simulink model "F104_FC2_sim"  (R2026b)
settings: Solver=ode45  StopTime=200  MaxStep=0.01  RelTol=1e-6  AbsTol=1e-8
undefined symbols (not defined in the file or in its folder): A, alt_m, B, C, D, pos_scale, thetae, V_ms, x0
libraries: aerolibsim3d x2, sim3dlib x1
settings Model: Creator=tensei  LastModifiedBy=tensei

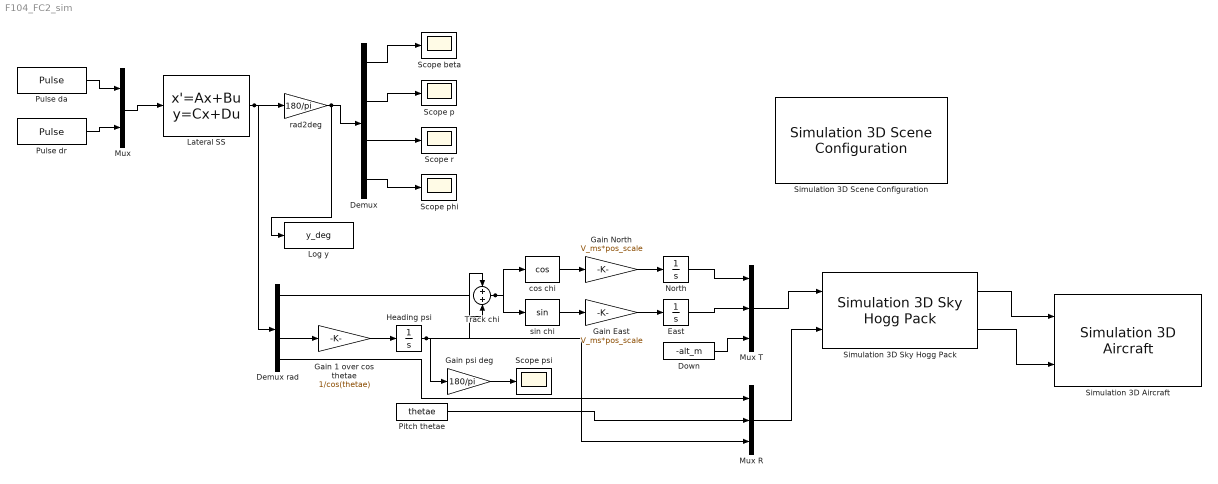
== system F104_FC2_sim ==
  Demux : Demux
  Demux rad : Demux
  Down : Constant  Value=-alt_m
  East : Integrator
  Gain 1 over cos thetae : Gain  Gain=1/cos(thetae)
  Gain East : Gain  Gain=V_ms*pos_scale
  Gain North : Gain  Gain=V_ms*pos_scale
  Gain psi deg : Gain  Gain=180/pi
  Heading psi : Integrator
  Lateral SS : StateSpace  A=A  B=B  C=C  D=D  InitialCondition=x0
  Log y : ToWorkspace  VariableName=y_deg  SampleTime=-1
  Mux : Mux  Inputs=2
  Mux R : Mux  Inputs=3
  Mux T : Mux  Inputs=3
  North : Integrator
  Pitch thetae : Constant  Value=thetae
  Pulse da : DiscretePulseGenerator  PulseType=Time based  Amplitude=0  Period=100
  Pulse dr : DiscretePulseGenerator  PulseType=Time based  Amplitude=0.034906  Period=100
  Scope beta : Scope
  Scope p : Scope
  Scope phi : Scope
  Scope psi : Scope
  Scope r : Scope
  Simulation 3D Aircraft : aerolibsim3d/Simulation 3D Aircraft  Priority=-1  Mesh=Sky Hogg  MeshPath=/MathWorksAerospaceContent/Vehicles/Aircraft/Custom/Mesh/SK_HL20.SK_HL20  MeshPathAT=/MathWorksAerospaceContent/Vehicles/Aircraft/AirTransport/Mesh/SK_AirTransport.SK_AirTransport  MeshPathGA=/MathWorksAerospaceContent/Vehicles/Aircraft/GeneralAviation/Mesh/SK_GeneralAviation.SK_GeneralAviation  AircraftColor=Red  ActorName=SimulinkVehicle1  ShowICs=on  Translation=[0 0 0; zeros(10,3)]  Rotation=[0 0 0; zeros(10,3)]  ScaleInputPort=Dialog  Scale=[1 1 1]  InitialScale=[1 1 1]  IsGHSensorEnabled=off  AreGHRaysVisible=off  IsOutputReshapeEnabled=off  GHRayLength=1524  GHBodyOffset=0.90  GHFrontTireRadius=0.21  GHLeftTireRadius=0.21  GHRightTireRadius=0.21  WoWSensorTolerance=0.05  LightsConfig=Automatic lights  LandingLightIntensity=300000  LandingLightConeAngle=15  CustomLeftLandingLightLocation=[0 0 0]  CustomLeftLandingLightOrientation=[0 0 0]  CustomRightLandingLightLocation=[0 0 0]  CustomRightLandingLightOrientation=[0 0 0]  TaxiLightIntensity=150000  TaxiLightConeAngle=36  CustomTaxiLightLocation=[0 0 0]  CustomTaxiLightOrientation=[0 0 0]  NavLightIntensity=500  PositionLightIntensity=500  StrobeLightIntensity=5000  WingtipStrobePeriod=1.5  WingtipStrobePulseWidth=6  TailStrobePeriod=1.5  TailStrobePulseWidth=6  BeaconLightIntensity=4000  BeaconPeriod=1.5  BeaconPulseWidth=10  SampleTime=-1  ActorType=SimulinkVehicle  ID=1  aMode=0  ActorTag=SimulinkVehicle1
  Simulation 3D Scene Configuration : sim3dlib/Simulation 3D Scene Configuration  Priority=0  EnableWindow=on  ViewerType=Default Viewer  ProjectFormat=Default Scenes  SceneDesc=Empty scene  ProjectName=/usr/local/MATLAB/R2026b/toolbox/shared/sim3d_projects/automotive_project_linux/UE/LinuxNoEditor/VehicleSimulation.sh  ScenePath=/Game/Maps/HwStrght  EnableOpenDRIVE=off  vehTagList={'Custom';'Scene Origin';'SimulinkVehicle1'}  vehTag=SimulinkVehicle1  AttachedCameraRelativeTranslation=[0 0 0]  FreeCameraDefaultInitialTranslation=[-6, 0, 2]  AttachedCameraRelativeRotation=[0, -15, 0]  FreeCameraDefaultInitialRotation=[0, -15, 0]  ViewpointName=Custom  FreeCameraInitialTranslation=[0, 0, 0]  FreeCameraInitialRotation=[0, 0, 0]  OpVisEn=off  Ts=.1  EnableRemoteAccess=off  SimulationMode=CoSimulation  SimulateUsing=Interpreted execution  EnableAnimationRecording=off  OverrideDefaultRecording=off  AnimationRecordingFileName=sim3dAnimation.mat  AnimationRecordingInterval=[0 inf]  EnableWeather=off  SunAzimuth=90  SunAltitude=40.0  EnableGeospatialSun=off  Latitude=0  Longitude=0  Date=2023-01-01  Time=10:30:00  GeoTimeZone=-5.0  SunDaylightSaving=off  wind=1  clouds=10  EnableVolumetricClouds=off  CloudCoverage=0  CloudAltitude=6  fog=0  rain=0  RaindropsEffect=off  SnowDensity=0  EnableGeospatial=off  TilesetSource=Earth terrain  UseTrueOrigin=off  OriginHeight=200  OriginLatitude=40.744652  OriginLongitude=-73.988864  MapStyle=Aerial  AdditionalAssetIDs=[]  UseAdvancedSunSky=off  SolarTime=11  TimeZone=-5  Day=21  Month=9  Year=2022  UseDaylightSavingTime=on  DSTStartDay=10  DSTStartMonth=3  DSTEndDay=3  DSTEndMonth=11  DSTSwitchHour=2  sensorTag=MainCamera1  sensorId=1  sensorName=MainCamera1  mountLoc=Origin  offsetFlag=off  tmountOffset=[0, 0, 0]  rmountOffset=[0, 0, 0]  HorizontalResolution=1280  VerticalResolution=720  HorizontalFOV=60  mountPoint=[0 0 0]  mountOrientation=[0 0 0]  aMode=5  ID=1  GeoTrigger=Inactive  ViewNameList={'Custom'}  ViewTranslationList={'[0 0 0]'}  ViewRotationList={'[0 0 0]'}
      settings: LibrarySourceBlock=sl3dlib/Simulation 3D/Environment/Simulation 3D Scene Configuration
  Simulation 3D Sky Hogg Pack : aerolibsim3d/Simulation 3D Sky Hogg Pack  Propeller_R=off  Rudder_R=off  Elevator_R=off  Left_Aileron_R=off  Right_Aileron_R=off  Flaps_R=off  Nose_Wheel_Strut_R=off  Nose_Wheel_R=off  Left_Wheel_R=off  Right_Wheel_R=off  EnableUETransform=on  GeoRadioButton=NED  EnableRotationOffset=off  RotationOffset=[0 0 0]
      settings: AttributesFormatString=NED
  Track chi : Sum
  cos chi : Trigonometry  Operator=cos
  rad2deg : Gain  Gain=180/pi
  sin chi : Trigonometry
  wires:
  Pulse da/1 -> Mux/1
  Pulse dr/1 -> Mux/2
  Mux/1 -> Lateral SS/1
  Lateral SS/1 -> rad2deg/1, Demux rad/1
  rad2deg/1 -> Demux/1, Log y/1
  Demux/1 -> Scope beta/1
  Demux/2 -> Scope p/1
  Demux/3 -> Scope r/1
  Demux/4 -> Scope phi/1
  Demux rad/3 -> Gain 1 over cos thetae/1
  Gain 1 over cos thetae/1 -> Heading psi/1
  Heading psi/1 -> Gain psi deg/1, Track chi/1, Mux R/3
  Gain psi deg/1 -> Scope psi/1
  Demux rad/1 -> Track chi/2
  Track chi/1 -> cos chi/1, sin chi/1
  cos chi/1 -> Gain North/1
  sin chi/1 -> Gain East/1
  Gain North/1 -> North/1
  Gain East/1 -> East/1
  North/1 -> Mux T/1
  East/1 -> Mux T/2
  Down/1 -> Mux T/3
  Demux rad/4 -> Mux R/1
  Pitch thetae/1 -> Mux R/2
  Mux T/1 -> Simulation 3D Sky Hogg Pack/1
  Mux R/1 -> Simulation 3D Sky Hogg Pack/2
  Simulation 3D Sky Hogg Pack/1 -> Simulation 3D Aircraft/1
  Simulation 3D Sky Hogg Pack/2 -> Simulation 3D Aircraft/2
